simulink model "dual_module"  (R2024b)
settings: Solver=VariableStepAuto  StartTime=0.0  StopTime=SIMULATION_TIME  MaxStep=1e-07  RelTol=1e-3
undefined symbols (not defined in the file or in its folder): bat_1, bat_2, battery_1_cutoff_time, battery_2_priority_to_zero, f_pi, P
libraries: fl_lib x15, nesl_utility x15, ee_lib x11, slpidlib x4, batteryecm_lib x2, simulink x1
(part 2 of 2)

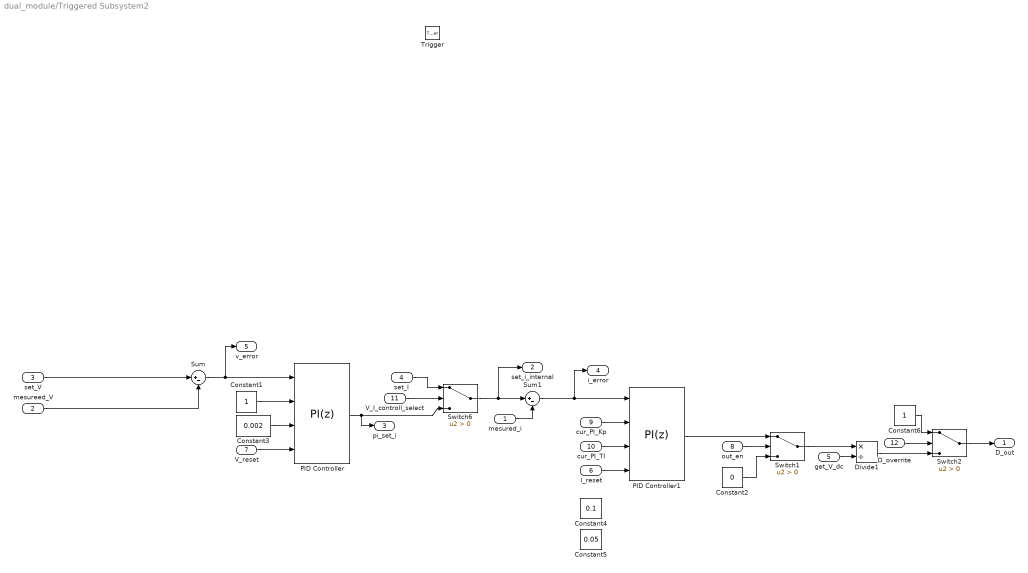
== system dual_module/Triggered Subsystem2 ==
  mesured_i : Inport  LatchByDelayingOutsideSignal=on
  mesureed_V : Inport  Port=2  LatchByDelayingOutsideSignal=on
  set_V : Inport  Port=3
  set_I : Inport  Port=4
  get_V_dc : Inport  Port=5
  I_reset : Inport  Port=6
  V_reset : Inport  Port=7
  out_en : Inport  Port=8
  cur_PI_Kp : Inport  Port=9
  cur_PI_TI : Inport  Port=10
  V_I_controll_select : Inport  Port=11
  D_overrite : Inport  Port=12
  Trigger : TriggerPort  TriggerType=falling  VariantControl=(inherit)
  Constant1 : Constant
  Constant2 : Constant  Value=0
  Constant3 : Constant  Value=0.002
  Constant4 : Constant  Value=0.1
  Constant5 : Constant  Value=0.05
  Constant6 : Constant
  Divide1 : Product  Inputs=*/
  PID Controller : slpidlib/PID Controller  Controller=PI  Form=Parallel  TimeDomain=Discrete-time  UseExternalTs=off  SampleTime=-1  IntegratorMethod=Forward Euler  FilterMethod=Forward Euler  ControllerParametersSource=external  P=0.6  I=50  UseKiTs=on  D=0  UseExternalDerivativeSource=off  N=100  UseFilter=on  TunerSelectOption=Transfer Function Based (PID Tuner App)  InitialConditionSource=internal  InitialConditionForIntegrator=0  InitialConditionForFilter=0  DifferentiatorICPrevScaledInput=0  ExternalReset=either  TrackingMode=off  Kt=1  LimitOutput=on  SatLimitsSource=internal  UpperSaturationLimit=25  LowerSaturationLimit=-5  LinearizeAsGain=on  AntiWindupMode=none  Kb=1  LimitIntegrator=off  UpperIntegratorSaturationLimit=inf  LowerIntegratorSaturationLimit=-inf  POutMin=[]  POutMax=[]  IOutMin=[]  IOutMax=[]  DOutMin=[]  DOutMax=[]  NOutMin=[]  NOutMax=[]  SumOutMin=[]  SumOutMax=[]  SaturationOutMin=[]  SaturationOutMax=[]  PParamMin=[]  PParamMax=[]  IParamMin=[]  IParamMax=[]  DParamMin=[]  DParamMax=[]  NParamMin=[]  NParamMax=[]  KbParamMin=[]  KbParamMax=[]  KtParamMin=[]  KtParamMax=[]  KbOutMin=[]  KbOutMax=[]  KtOutMin=[]  KtOutMax=[]  IntegratorOutMin=[]  IntegratorOutMax=[]  FilterOutMin=[]  FilterOutMax=[]  SumI1OutMin=[]  SumI1OutMax=[]  SumI2OutMin=[]  SumI2OutMax=[]  SumI3OutMin=[]  SumI3OutMax=[]  SumI4OutMin=[]  SumI4OutMax=[]  SumDOutMin=[]  SumDOutMax=[]  DifferentiatorOutMin=[]  DifferentiatorOutMax=[]  FilterDiffOutCoefMin=[]  FilterDiffOutCoefMax=[]  ReciprocalOutMin=[]  ReciprocalOutMax=[]  SumDenOutMin=[]  SumDenOutMax=[]  SumNumOutMin=[]  SumNumOutMax=[]  DivideOutMin=[]  DivideOutMax=[]  UdiffTsProdOutMin=[]  UdiffTsProdOutMax=[]  NTsProdOutMin=[]  NTsProdOutMax=[]  UintegralTsProdOutMin=[]  UintegralTsProdOutMax=[]  UngainTsProdOutMin=[]  UngainTsProdOutMax=[]  ClampingZeroOutDataTypeStr=Inherit: Inherit via back propagation  ClampingZeroOutMin=[]  ClampingZeroOutMax=[]  FilterDenConstantOutDataTypeStr=Inherit: Inherit via back propagation  FilterDenConstantOutMin=[]  FilterDenConstantOutMax=[]  PCopyOutDataTypeStr=Inherit: Inherit via back propagation  PCopyOutMin=[]  PCopyOutMax=[]  NCopyOutDataTypeStr=Inherit: Inherit via back propagation  NCopyOutMin=[]  NCopyOutMax=[]  IntegratorContinuousStateAttributes=''  IntegratorStateMustResolveToSignalObject=off  IntegratorRTWStateStorageClass=Auto  FilterContinuousStateAttributes=''  FilterStateMustResolveToSignalObject=off  FilterRTWStateStorageClass=Auto  ParallelPVariant=ExternalParameters  IdealPVariant=Disabled  IVariant=ExternalParameters  DVariant=Disabled  IntegratorVariant=Discrete  SatVariant=Enabled  AWVariant=Passthrough  PCopyVariant=Disabled  TRVariant=Disabled  FdbkBlocksVariant=Forward  IdealPFdbkVariant=Disabled  SatFdbkVariant=Disabled  DerivativeFilterVariant=Disabled  NVariant=Disabled  NCopyVariant=Disabled_SignalSpec  FilterICVariant=Disabled  IntegratorICVariant=InternalICs  ExternalResetVariant=ExternalReset  TRSumVariant=Passthrough  SumFdbkVariant=Disabled  SumVariant=Sum_PI  TsampFilterVariant=InternalTs  TsampNgainVariant=Passthrough  TsampIntegralVariant=Disabled_SignalSpec  ExternalSaturationOutDataTypeStr=Inherit: Same as second input  DerivativeSourceVariant=Disabled  PreIntVariant=InternalPreInt
  PID Controller1 : slpidlib/PID Controller  Controller=PI  Form=Parallel  TimeDomain=Discrete-time  UseExternalTs=off  SampleTime=-1  IntegratorMethod=Forward Euler  FilterMethod=Forward Euler  ControllerParametersSource=external  P=0.6  I=0.1  UseKiTs=on  D=0  UseExternalDerivativeSource=off  N=100  UseFilter=on  TunerSelectOption=Transfer Function Based (PID Tuner App)  InitialConditionSource=internal  InitialConditionForIntegrator=0  InitialConditionForFilter=0  DifferentiatorICPrevScaledInput=0  ExternalReset=either  TrackingMode=off  Kt=1  LimitOutput=on  SatLimitsSource=internal  UpperSaturationLimit=23  LowerSaturationLimit=0  LinearizeAsGain=on  AntiWindupMode=clamping  Kb=1  LimitIntegrator=off  UpperIntegratorSaturationLimit=inf  LowerIntegratorSaturationLimit=-inf  POutMin=[]  POutMax=[]  IOutMin=[]  IOutMax=[]  DOutMin=[]  DOutMax=[]  NOutMin=[]  NOutMax=[]  SumOutMin=[]  SumOutMax=[]  SaturationOutMin=[]  SaturationOutMax=[]  PParamMin=[]  PParamMax=[]  IParamMin=[]  IParamMax=[]  DParamMin=[]  DParamMax=[]  NParamMin=[]  NParamMax=[]  KbParamMin=[]  KbParamMax=[]  KtParamMin=[]  KtParamMax=[]  KbOutMin=[]  KbOutMax=[]  KtOutMin=[]  KtOutMax=[]  IntegratorOutMin=[]  IntegratorOutMax=[]  FilterOutMin=[]  FilterOutMax=[]  SumI1OutMin=[]  SumI1OutMax=[]  SumI2OutMin=[]  SumI2OutMax=[]  SumI3OutMin=[]  SumI3OutMax=[]  SumI4OutMin=[]  SumI4OutMax=[]  SumDOutMin=[]  SumDOutMax=[]  DifferentiatorOutMin=[]  DifferentiatorOutMax=[]  FilterDiffOutCoefMin=[]  FilterDiffOutCoefMax=[]  ReciprocalOutMin=[]  ReciprocalOutMax=[]  SumDenOutMin=[]  SumDenOutMax=[]  SumNumOutMin=[]  SumNumOutMax=[]  DivideOutMin=[]  DivideOutMax=[]  UdiffTsProdOutMin=[]  UdiffTsProdOutMax=[]  NTsProdOutMin=[]  NTsProdOutMax=[]  UintegralTsProdOutMin=[]  UintegralTsProdOutMax=[]  UngainTsProdOutMin=[]  UngainTsProdOutMax=[]  ClampingZeroOutDataTypeStr=Inherit: Inherit via back propagation  ClampingZeroOutMin=[]  ClampingZeroOutMax=[]  FilterDenConstantOutDataTypeStr=Inherit: Inherit via back propagation  FilterDenConstantOutMin=[]  FilterDenConstantOutMax=[]  PCopyOutDataTypeStr=Inherit: Inherit via back propagation  PCopyOutMin=[]  PCopyOutMax=[]  NCopyOutDataTypeStr=Inherit: Inherit via back propagation  NCopyOutMin=[]  NCopyOutMax=[]  IntegratorContinuousStateAttributes=''  IntegratorStateMustResolveToSignalObject=off  IntegratorRTWStateStorageClass=Auto  FilterContinuousStateAttributes=''  FilterStateMustResolveToSignalObject=off  FilterRTWStateStorageClass=Auto  ParallelPVariant=ExternalParameters  IdealPVariant=Disabled  IVariant=ExternalParameters  DVariant=Disabled  IntegratorVariant=Discrete  SatVariant=Enabled  AWVariant=DiscClampingParallel  PCopyVariant=Disabled  TRVariant=Disabled  FdbkBlocksVariant=Forward  IdealPFdbkVariant=Disabled  SatFdbkVariant=Disabled  DerivativeFilterVariant=Disabled  NVariant=Disabled  NCopyVariant=Disabled_SignalSpec  FilterICVariant=Disabled  IntegratorICVariant=InternalICs  ExternalResetVariant=ExternalReset  TRSumVariant=Passthrough  SumFdbkVariant=Disabled  SumVariant=Sum_PI  TsampFilterVariant=InternalTs  TsampNgainVariant=Passthrough  TsampIntegralVariant=Disabled_SignalSpec  ExternalSaturationOutDataTypeStr=Inherit: Same as second input  DerivativeSourceVariant=Disabled  PreIntVariant=InternalPreInt
  Sum : Sum  Inputs=|+-
  Sum1 : Sum  Inputs=|+-
  Switch1 : Switch  Criteria=u2 > Threshold  SaturateOnIntegerOverflow=off  InputSameDT=off
  Switch2 : Switch  Criteria=u2 > Threshold  SaturateOnIntegerOverflow=off  InputSameDT=off
  Switch6 : Switch  Criteria=u2 > Threshold  SaturateOnIntegerOverflow=off  InputSameDT=off
  D_out : Outport
  set_i_internal : Outport  Port=2
  pi_set_i : Outport  Port=3
  i_error : Outport  Port=4
  v_error : Outport  Port=5
  wires:
  get_V_dc/1 -> Divide1/2
  Switch1/1 -> Divide1/1
  mesured_i/1 -> Sum1/2
  Sum1/1 -> i_error/1, PID Controller1/1
  Sum/1 -> PID Controller/1, v_error/1
  Constant1/1 -> PID Controller/2
  Constant3/1 -> PID Controller/3
  Switch6/1 -> set_i_internal/1, Sum1/1
  PID Controller/1 -> Switch6/3, pi_set_i/1
  set_I/1 -> Switch6/1
  set_V/1 -> Sum/1
  mesureed_V/1 -> Sum/2
  V_reset/1 -> PID Controller/4
  I_reset/1 -> PID Controller1/4
  out_en/1 -> Switch1/2
  cur_PI_Kp/1 -> PID Controller1/2
  cur_PI_TI/1 -> PID Controller1/3
  V_I_controll_select/1 -> Switch6/2
  Constant6/1 -> Switch2/1
  Divide1/1 -> Switch2/3
  Switch2/1 -> D_out/1
  D_overrite/1 -> Switch2/2
  Constant2/1 -> Switch1/3
  PID Controller1/1 -> Switch1/1

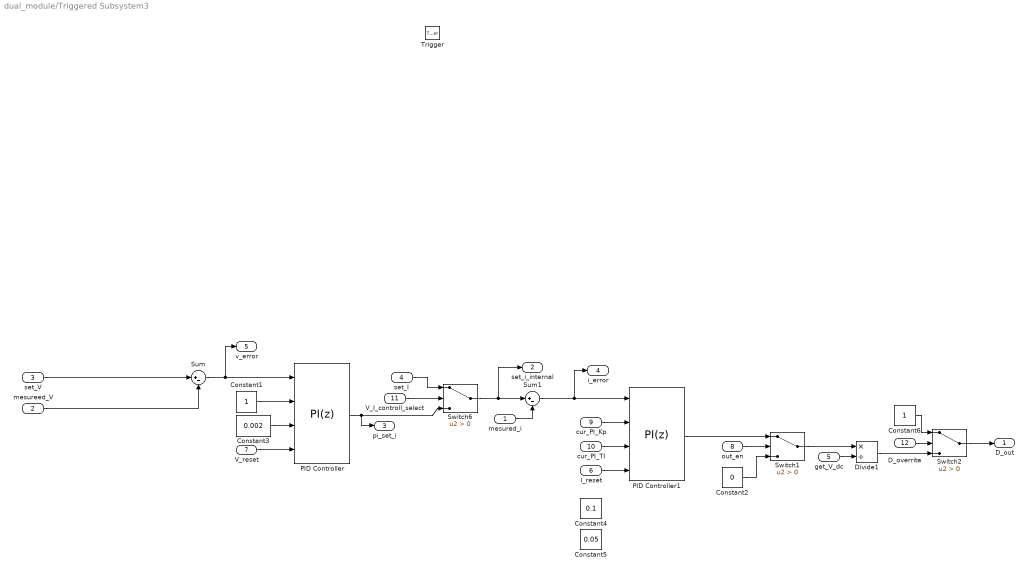
== system dual_module/Triggered Subsystem3 ==
  mesured_i : Inport  LatchByDelayingOutsideSignal=on
  mesureed_V : Inport  Port=2  LatchByDelayingOutsideSignal=on
  set_V : Inport  Port=3
  set_I : Inport  Port=4
  get_V_dc : Inport  Port=5
  I_reset : Inport  Port=6
  V_reset : Inport  Port=7
  out_en : Inport  Port=8
  cur_PI_Kp : Inport  Port=9
  cur_PI_TI : Inport  Port=10
  V_I_controll_select : Inport  Port=11
  D_overrite : Inport  Port=12
  Trigger : TriggerPort  TriggerType=falling  VariantControl=(inherit)
  Constant1 : Constant
  Constant2 : Constant  Value=0
  Constant3 : Constant  Value=0.002
  Constant4 : Constant  Value=0.1
  Constant5 : Constant  Value=0.05
  Constant6 : Constant
  Divide1 : Product  Inputs=*/
  PID Controller : slpidlib/PID Controller  Controller=PI  Form=Parallel  TimeDomain=Discrete-time  UseExternalTs=off  SampleTime=-1  IntegratorMethod=Forward Euler  FilterMethod=Forward Euler  ControllerParametersSource=external  P=0.6  I=50  UseKiTs=on  D=0  UseExternalDerivativeSource=off  N=100  UseFilter=on  TunerSelectOption=Transfer Function Based (PID Tuner App)  InitialConditionSource=internal  InitialConditionForIntegrator=0  InitialConditionForFilter=0  DifferentiatorICPrevScaledInput=0  ExternalReset=either  TrackingMode=off  Kt=1  LimitOutput=on  SatLimitsSource=internal  UpperSaturationLimit=25  LowerSaturationLimit=-5  LinearizeAsGain=on  AntiWindupMode=none  Kb=1  LimitIntegrator=off  UpperIntegratorSaturationLimit=inf  LowerIntegratorSaturationLimit=-inf  POutMin=[]  POutMax=[]  IOutMin=[]  IOutMax=[]  DOutMin=[]  DOutMax=[]  NOutMin=[]  NOutMax=[]  SumOutMin=[]  SumOutMax=[]  SaturationOutMin=[]  SaturationOutMax=[]  PParamMin=[]  PParamMax=[]  IParamMin=[]  IParamMax=[]  DParamMin=[]  DParamMax=[]  NParamMin=[]  NParamMax=[]  KbParamMin=[]  KbParamMax=[]  KtParamMin=[]  KtParamMax=[]  KbOutMin=[]  KbOutMax=[]  KtOutMin=[]  KtOutMax=[]  IntegratorOutMin=[]  IntegratorOutMax=[]  FilterOutMin=[]  FilterOutMax=[]  SumI1OutMin=[]  SumI1OutMax=[]  SumI2OutMin=[]  SumI2OutMax=[]  SumI3OutMin=[]  SumI3OutMax=[]  SumI4OutMin=[]  SumI4OutMax=[]  SumDOutMin=[]  SumDOutMax=[]  DifferentiatorOutMin=[]  DifferentiatorOutMax=[]  FilterDiffOutCoefMin=[]  FilterDiffOutCoefMax=[]  ReciprocalOutMin=[]  ReciprocalOutMax=[]  SumDenOutMin=[]  SumDenOutMax=[]  SumNumOutMin=[]  SumNumOutMax=[]  DivideOutMin=[]  DivideOutMax=[]  UdiffTsProdOutMin=[]  UdiffTsProdOutMax=[]  NTsProdOutMin=[]  NTsProdOutMax=[]  UintegralTsProdOutMin=[]  UintegralTsProdOutMax=[]  UngainTsProdOutMin=[]  UngainTsProdOutMax=[]  ClampingZeroOutDataTypeStr=Inherit: Inherit via back propagation  ClampingZeroOutMin=[]  ClampingZeroOutMax=[]  FilterDenConstantOutDataTypeStr=Inherit: Inherit via back propagation  FilterDenConstantOutMin=[]  FilterDenConstantOutMax=[]  PCopyOutDataTypeStr=Inherit: Inherit via back propagation  PCopyOutMin=[]  PCopyOutMax=[]  NCopyOutDataTypeStr=Inherit: Inherit via back propagation  NCopyOutMin=[]  NCopyOutMax=[]  IntegratorContinuousStateAttributes=''  IntegratorStateMustResolveToSignalObject=off  IntegratorRTWStateStorageClass=Auto  FilterContinuousStateAttributes=''  FilterStateMustResolveToSignalObject=off  FilterRTWStateStorageClass=Auto  ParallelPVariant=ExternalParameters  IdealPVariant=Disabled  IVariant=ExternalParameters  DVariant=Disabled  IntegratorVariant=Discrete  SatVariant=Enabled  AWVariant=Passthrough  PCopyVariant=Disabled  TRVariant=Disabled  FdbkBlocksVariant=Forward  IdealPFdbkVariant=Disabled  SatFdbkVariant=Disabled  DerivativeFilterVariant=Disabled  NVariant=Disabled  NCopyVariant=Disabled_SignalSpec  FilterICVariant=Disabled  IntegratorICVariant=InternalICs  ExternalResetVariant=ExternalReset  TRSumVariant=Passthrough  SumFdbkVariant=Disabled  SumVariant=Sum_PI  TsampFilterVariant=InternalTs  TsampNgainVariant=Passthrough  TsampIntegralVariant=Disabled_SignalSpec  ExternalSaturationOutDataTypeStr=Inherit: Same as second input  DerivativeSourceVariant=Disabled  PreIntVariant=InternalPreInt
  PID Controller1 : slpidlib/PID Controller  Controller=PI  Form=Parallel  TimeDomain=Discrete-time  UseExternalTs=off  SampleTime=-1  IntegratorMethod=Forward Euler  FilterMethod=Forward Euler  ControllerParametersSource=external  P=0.6  I=0.1  UseKiTs=on  D=0  UseExternalDerivativeSource=off  N=100  UseFilter=on  TunerSelectOption=Transfer Function Based (PID Tuner App)  InitialConditionSource=internal  InitialConditionForIntegrator=0  InitialConditionForFilter=0  DifferentiatorICPrevScaledInput=0  ExternalReset=either  TrackingMode=off  Kt=1  LimitOutput=on  SatLimitsSource=internal  UpperSaturationLimit=23  LowerSaturationLimit=0  LinearizeAsGain=on  AntiWindupMode=clamping  Kb=1  LimitIntegrator=off  UpperIntegratorSaturationLimit=inf  LowerIntegratorSaturationLimit=-inf  POutMin=[]  POutMax=[]  IOutMin=[]  IOutMax=[]  DOutMin=[]  DOutMax=[]  NOutMin=[]  NOutMax=[]  SumOutMin=[]  SumOutMax=[]  SaturationOutMin=[]  SaturationOutMax=[]  PParamMin=[]  PParamMax=[]  IParamMin=[]  IParamMax=[]  DParamMin=[]  DParamMax=[]  NParamMin=[]  NParamMax=[]  KbParamMin=[]  KbParamMax=[]  KtParamMin=[]  KtParamMax=[]  KbOutMin=[]  KbOutMax=[]  KtOutMin=[]  KtOutMax=[]  IntegratorOutMin=[]  IntegratorOutMax=[]  FilterOutMin=[]  FilterOutMax=[]  SumI1OutMin=[]  SumI1OutMax=[]  SumI2OutMin=[]  SumI2OutMax=[]  SumI3OutMin=[]  SumI3OutMax=[]  SumI4OutMin=[]  SumI4OutMax=[]  SumDOutMin=[]  SumDOutMax=[]  DifferentiatorOutMin=[]  DifferentiatorOutMax=[]  FilterDiffOutCoefMin=[]  FilterDiffOutCoefMax=[]  ReciprocalOutMin=[]  ReciprocalOutMax=[]  SumDenOutMin=[]  SumDenOutMax=[]  SumNumOutMin=[]  SumNumOutMax=[]  DivideOutMin=[]  DivideOutMax=[]  UdiffTsProdOutMin=[]  UdiffTsProdOutMax=[]  NTsProdOutMin=[]  NTsProdOutMax=[]  UintegralTsProdOutMin=[]  UintegralTsProdOutMax=[]  UngainTsProdOutMin=[]  UngainTsProdOutMax=[]  ClampingZeroOutDataTypeStr=Inherit: Inherit via back propagation  ClampingZeroOutMin=[]  ClampingZeroOutMax=[]  FilterDenConstantOutDataTypeStr=Inherit: Inherit via back propagation  FilterDenConstantOutMin=[]  FilterDenConstantOutMax=[]  PCopyOutDataTypeStr=Inherit: Inherit via back propagation  PCopyOutMin=[]  PCopyOutMax=[]  NCopyOutDataTypeStr=Inherit: Inherit via back propagation  NCopyOutMin=[]  NCopyOutMax=[]  IntegratorContinuousStateAttributes=''  IntegratorStateMustResolveToSignalObject=off  IntegratorRTWStateStorageClass=Auto  FilterContinuousStateAttributes=''  FilterStateMustResolveToSignalObject=off  FilterRTWStateStorageClass=Auto  ParallelPVariant=ExternalParameters  IdealPVariant=Disabled  IVariant=ExternalParameters  DVariant=Disabled  IntegratorVariant=Discrete  SatVariant=Enabled  AWVariant=DiscClampingParallel  PCopyVariant=Disabled  TRVariant=Disabled  FdbkBlocksVariant=Forward  IdealPFdbkVariant=Disabled  SatFdbkVariant=Disabled  DerivativeFilterVariant=Disabled  NVariant=Disabled  NCopyVariant=Disabled_SignalSpec  FilterICVariant=Disabled  IntegratorICVariant=InternalICs  ExternalResetVariant=ExternalReset  TRSumVariant=Passthrough  SumFdbkVariant=Disabled  SumVariant=Sum_PI  TsampFilterVariant=InternalTs  TsampNgainVariant=Passthrough  TsampIntegralVariant=Disabled_SignalSpec  ExternalSaturationOutDataTypeStr=Inherit: Same as second input  DerivativeSourceVariant=Disabled  PreIntVariant=InternalPreInt
  Sum : Sum  Inputs=|+-
  Sum1 : Sum  Inputs=|+-
  Switch1 : Switch  Criteria=u2 > Threshold  SaturateOnIntegerOverflow=off  InputSameDT=off
  Switch2 : Switch  Criteria=u2 > Threshold  SaturateOnIntegerOverflow=off  InputSameDT=off
  Switch6 : Switch  Criteria=u2 > Threshold  SaturateOnIntegerOverflow=off  InputSameDT=off
  D_out : Outport
  set_i_internal : Outport  Port=2
  pi_set_i : Outport  Port=3
  i_error : Outport  Port=4
  v_error : Outport  Port=5
  wires:
  D_overrite/1 -> Switch2/2
  Switch2/1 -> D_out/1
  Divide1/1 -> Switch2/3
  Constant6/1 -> Switch2/1
  V_I_controll_select/1 -> Switch6/2
  cur_PI_TI/1 -> PID Controller1/3
  cur_PI_Kp/1 -> PID Controller1/2
  out_en/1 -> Switch1/2
  I_reset/1 -> PID Controller1/4
  V_reset/1 -> PID Controller/4
  mesureed_V/1 -> Sum/2
  set_V/1 -> Sum/1
  set_I/1 -> Switch6/1
  PID Controller/1 -> pi_set_i/1, Switch6/3
  Switch6/1 -> Sum1/1, set_i_internal/1
  Constant3/1 -> PID Controller/3
  Constant1/1 -> PID Controller/2
  Sum/1 -> v_error/1, PID Controller/1
  Sum1/1 -> PID Controller1/1, i_error/1
  mesured_i/1 -> Sum1/2
  Switch1/1 -> Divide1/1
  get_V_dc/1 -> Divide1/2
  Constant2/1 -> Switch1/3
  PID Controller1/1 -> Switch1/1

== matlab function dual_module/MATLAB Function ==
  data: V_set output; reset_I output; reset_V output; out_en output; cur_PI_Kp output; cur_PI_Ti output; V_I_controll_select output; D_1_overrite output; state_out output; state input; priority input; D_loopback input; v_0 input; i_0 input; V_dc input; I_out input; V_out input; priority_0_module_V_0 input; state_from_Priority_0 input
function [V_set, reset_I, reset_V, out_en,cur_PI_Kp, cur_PI_Ti, V_I_controll_select,D_1_overrite, state_out]= PI_state_machine(state, priority, D_loopback, v_0, i_0, V_dc, I_out, V_out, priority_0_module_V_0, state_from_Priority_0)

    V_set               = 0;
    reset_I             = 0;
    reset_V             = 0;
    out_en              = 0;
    cur_PI_Kp           = 0;
    cur_PI_Ti           = 0;
    V_I_controll_select = 0;
    D_1_overrite        = 0;
    state_out           = state;


    persistent p_reset_I;
    persistent p_reset_V;
    persistent fast_charging;

    if isempty(p_reset_I)
        p_reset_I = 0;
    end
    if isempty(p_reset_V)
        p_reset_V = 0;
    end
    if isempty(fast_charging)
        fast_charging = 0;
    end

    switch state
        case 0 % idle
            cur_PI_Kp           = 0;
            cur_PI_Ti           = 0;
            out_en              = 0;
            V_set               = 0;
            V_I_controll_select = 0;
            D_1_overrite        = 0;

            if priority == 0
                state_out = 1; % to first charge
            elseif (priority == 1) && (state_from_Priority_0 == 5)
                state_out = 2; % to fallback state
            end

        case 1 % first charge

            target_V = V_dc + 1; % so the D has to saturate at some point
            if v_0 > 0.9 * target_V
                fast_charging = 0;
                p_reset_I = 1 - p_reset_I;
                p_reset_V = 1 - p_reset_V;
            elseif v_0 < 0.3 * target_V
                fast_charging = 1;
            end % fast cap charging flip flop

            if fast_charging == 1
                V_I_controll_select = 1;
            else
                V_I_controll_select = 0;
            end

            V_set        = target_V;
            cur_PI_Kp    = 0.1;
            cur_PI_Ti    = 0.05;
            D_1_overrite = 0;
            out_en       = 1;

            if D_loopback >= 0.95
                state_out = 5;
            end


        case 2 % charge to a fallback voltage
            target_V = priority_0_module_V_0 - 0.5; % so the voltage dont overshoot and be drained of current too quickly
            if (v_0 > 0.9 * target_V) && (fast_charging == 1)
                fast_charging = 0;
                p_reset_I = 1 - p_reset_I;
                p_reset_V = 1 - p_reset_V;
            elseif v_0 < 0.3 * target_V
                fast_charging = 1;
            end % fast cap charging flip flop

            if fast_charging == 1
                V_I_controll_select = 1;
            else
                V_I_controll_select = 0;
            end

            V_set        = target_V;
            cur_PI_Kp    = 0.05;
            cur_PI_Ti    = 0.05;
            out_en       = 1;
            D_1_overrite = 0;

            if v_0 >= target_V
                p_reset_I = 1 - p_reset_I;
                p_reset_V = 1 - p_reset_V;
                state_out = 3;
            end


        case 3 % fallback hold
            target_V            = priority_0_module_V_0 - 0.5;
            V_set               = target_V;
            cur_PI_Kp           = 0.1;
            cur_PI_Ti           = 0.05;
            out_en              = 1;
            V_I_controll_select = 0;
            D_1_overrite        = 0;

            if priority == 0
                state_out = 4;
            end

        case 4 % charging up to full cycle
            target_V            = V_dc + 1;
            V_set               = target_V;
            cur_PI_Kp           = 0.3;
            cur_PI_Ti           = 0.15;
            out_en              = 1;
            V_I_controll_select = 0;
            D_1_overrite        = 0;
            if D_loopback > 0.95
                state_out = 5;
            end

        case 5 % 100% cycle
            D_1_overrite        = 1;
            cur_PI_Kp           = 0;
            cur_PI_Ti           = 0;
            out_en              = 1;
            V_set               = 0;
            V_I_controll_select = 0;
            if (i_0 < 0.1 * I_out) && (v_0 < 0.9 * V_out)
                state_out = 6;
            end


        case 6 % EOL
            out_en              = 0;
            V_set               = 0;
            cur_PI_Kp           = 0;
            cur_PI_Ti           = 0;
            V_I_controll_select = 0;
            D_1_overrite        = 0;
            if v_0 < 1
                state_out = 0;
            end

        otherwise
            cur_PI_Kp           = 0;
            cur_PI_Ti           = 0;
            out_en              = 0;
            state_out           = 0;
            V_set               = 0;
            V_I_controll_select = 0;
            D_1_overrite        = 0;
    end
    reset_I = p_reset_I;
    reset_V = p_reset_V;

== matlab function dual_module/MATLAB Function1 ==
  data: V_set output; reset_I output; reset_V output; out_en output; cur_PI_Kp output; cur_PI_Ti output; V_I_controll_select output; D_1_overrite output; state_out output; state input; priority input; D_loopback input; v_0 input; i_0 input; V_dc input; I_out input; V_out input; priority_0_module_V_0 input; state_from_Priority_0 input
function [V_set, reset_I, reset_V, out_en,cur_PI_Kp, cur_PI_Ti, V_I_controll_select,D_1_overrite, state_out]= PI_state_machine(state, priority, D_loopback, v_0, i_0, V_dc, I_out, V_out, priority_0_module_V_0, state_from_Priority_0)

    V_set               = 0;
    reset_I             = 0;
    reset_V             = 0;
    out_en              = 0;
    cur_PI_Kp           = 0;
    cur_PI_Ti           = 0;
    V_I_controll_select = 0;
    D_1_overrite        = 0;
    state_out           = state;


    persistent p_reset_I;
    persistent p_reset_V;
    persistent fast_charging;

    if isempty(p_reset_I)
        p_reset_I = 0;
    end
    if isempty(p_reset_V)
        p_reset_V = 0;
    end
    if isempty(fast_charging)
        fast_charging = 0;
    end

    switch state
        case 0 % idle
            cur_PI_Kp           = 0;
            cur_PI_Ti           = 0;
            out_en              = 0;
            V_set               = 0;
            V_I_controll_select = 0;
            D_1_overrite        = 0;

            if priority == 0
                state_out = 1; % to first charge
            elseif (priority == 1) && (state_from_Priority_0 == 5)
                state_out = 2; % to fallback state
            end

        case 1 % first charge

            target_V = V_dc + 1; % so the D has to saturate at some point
            if v_0 > 0.9 * target_V
                fast_charging = 0;
                p_reset_I = 1 - p_reset_I;
                p_reset_V = 1 - p_reset_V;
            elseif v_0 < 0.3 * target_V
                fast_charging = 1;
            end % fast cap charging flip flop

            if fast_charging == 1
                V_I_controll_select = 1;
            else
                V_I_controll_select = 0;
            end

            V_set        = target_V;
            cur_PI_Kp    = 0.1;
            cur_PI_Ti    = 0.05;
            D_1_overrite = 0;
            out_en       = 1;

            if D_loopback >= 0.95
                state_out = 5;
            end


        case 2 % charge to a fallback voltage
            target_V = priority_0_module_V_0 - 0.5; % so the voltage dont overshoot and be drained of current too quickly
            if (v_0 > 0.9 * target_V) && (fast_charging == 1)
                fast_charging = 0;
                p_reset_I = 1 - p_reset_I;
                p_reset_V = 1 - p_reset_V;
            elseif v_0 < 0.3 * target_V
                fast_charging = 1;
            end % fast cap charging flip flop

            if fast_charging == 1
                V_I_controll_select = 1;
            else
                V_I_controll_select = 0;
            end

            V_set        = target_V;
            cur_PI_Kp    = 0.05;
            cur_PI_Ti    = 0.05;
            out_en       = 1;
            D_1_overrite = 0;

            if v_0 >= target_V
                p_reset_I = 1 - p_reset_I;
                p_reset_V = 1 - p_reset_V;
                state_out = 3;
            end


        case 3 % fallback hold
            target_V            = priority_0_module_V_0 - 0.5;
            V_set               = target_V;
            cur_PI_Kp           = 0.1;
            cur_PI_Ti           = 0.05;
            out_en              = 1;
            V_I_controll_select = 0;
            D_1_overrite        = 0;

            if priority == 0
                state_out = 4;
            end

        case 4 % charging up to full cycle
            target_V            = V_dc + 1;
            V_set               = target_V;
            cur_PI_Kp           = 0.3;
            cur_PI_Ti           = 0.15;
            out_en              = 1;
            V_I_controll_select = 0;
            D_1_overrite        = 0;
            if D_loopback > 0.95
                state_out = 5;
            end

        case 5 % 100% cycle
            D_1_overrite        = 1;
            cur_PI_Kp           = 0;
            cur_PI_Ti           = 0;
            out_en              = 1;
            V_set               = 0;
            V_I_controll_select = 0;
            if (i_0 < 0.1 * I_out) && (v_0 < 0.9 * V_out)
                state_out = 6;
            end


        case 6 % EOL
            out_en              = 0;
            V_set               = 0;
            cur_PI_Kp           = 0;
            cur_PI_Ti           = 0;
            V_I_controll_select = 0;
            D_1_overrite        = 0;
            if v_0 < 1
                state_out = 0;
            end

        otherwise
            cur_PI_Kp           = 0;
            cur_PI_Ti           = 0;
            out_en              = 0;
            state_out           = 0;
            V_set               = 0;
            V_I_controll_select = 0;
            D_1_overrite        = 0;
    end
    reset_I = p_reset_I;
    reset_V = p_reset_V;
